simulink model "BESS_PV_WIND_STAGE2_R2_1_READABLE"  (R2026a)
settings: Solver=ode23t  StopTime=1.2  MaxStep=1e-5
InitFcn:
  | run(fullfile(fileparts(get_param(bdroot,'FileName')),'..','scripts','init_bess_pv_wind_stage2_r1.m'));
undefined symbols (not defined in the file): Control, G, S1, S2, S21, S2_API, W1
libraries: ee_lib x27, nesl_utility x23, fl_lib x10, simulink x4, sl_discontinuities x1
(part 2 of 2)

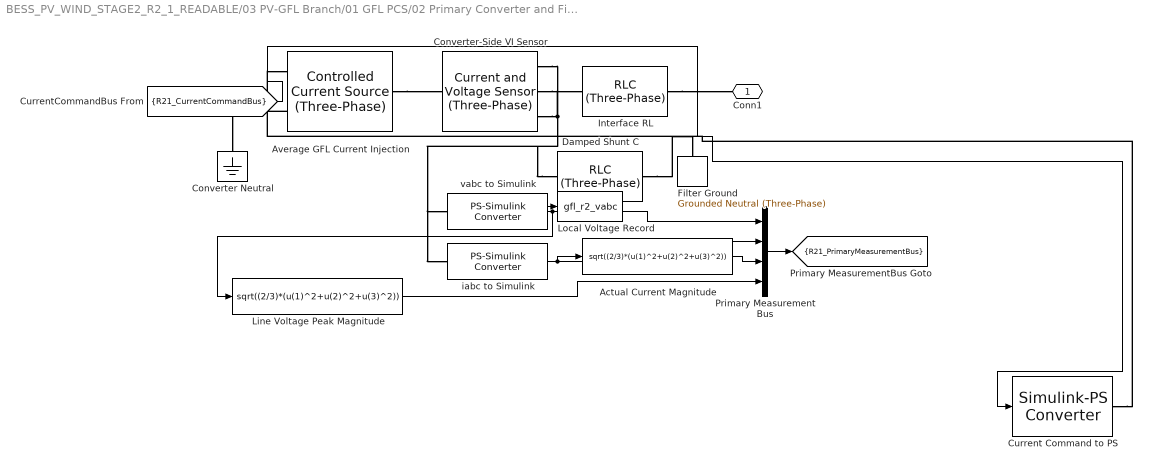
== system BESS_PV_WIND_STAGE2_R2_1_READABLE/03 PV-GFL Branch/01 GFL PCS/02 Primary Converter and Filter ==
  Actual Current Magnitude : Fcn  Expr=sqrt((2/3)*(u(1)^2+u(2)^2+u(3)^2))
  Average GFL Current Injection : ee_lib/Sources/Controlled Current Source (Three-Phase)  port_option=ee.enum.threePhasePort.composite  input_option=ee.enum.inputType.instantaneous  FRated=S1.base.f_Hz Hz  G_parasitic=1e-6 1/Ohm
  Converter Neutral : fl_lib/Electrical/Electrical Elements/Electrical Reference
  Converter-Side VI Sensor : ee_lib/Sensors & Transducers/Current and Voltage Sensor (Three-Phase)  port_option=ee.enum.threePhasePort.composite  vMeasurementType=ee.enum.vmeasurement.ll  outputUnit=ee.enum.unit.si  SRated=100e6 A*V  VRated=24e3 V  I_specify=off  I_priority=None  I=[0, 0, 0] A  I_nominal_specify=off  I_nominal_value=1  I_nominal_unit=A  V_specify=off  V_priority=None  V=[0, 0, 0] V  V_nominal_specify=off  V_nominal_value=1  V_nominal_unit=V
  Current Command to PS : nesl_utility/Simulink-PS Converter  PhysicalDomain=network_engine_domain  SubClassName=ps_input  LeftPortType=input  RightPortType=output  PseudoPeriodic=off  Frequencies=[]  NoiseDistribution=none  NoiseParameters=[]  Unit=A  AffineConversion=off  FilteringAndDerivatives=zero  SimscapeFilterOrder=1  InputFilterTimeConstant=0.001  UdotUserProvided=0
  Damped Shunt C : ee_lib/Passive/RLC Assemblies/RLC (Three-Phase)  port_option=ee.enum.threePhasePort.composite  component_structure=ee.enum.rlc.structure.SeriesRC  R=S1.filter.Rd_ohm Ohm  L=1e-3 H  C=S1.filter.C_F F  R_parasitic=0 Ohm  G_parasitic=0 1/Ohm  IL_specify=off  IL_priority=High  IL=[0, 0, 0] A  IL_nominal_specify=off  IL_nominal_value=1  IL_nominal_unit=A  VC_specify=off  VC_priority=High  VC=[0, 0, 0] V  VC_nominal_specify=off  VC_nominal_value=1  VC_nominal_unit=V
  Filter Ground : ee_lib/Connectors & References/Grounded Neutral (Three-Phase)  port_option=ee.enum.threePhasePort.composite
  Interface RL : ee_lib/Passive/RLC Assemblies/RLC (Three-Phase)  port_option=ee.enum.threePhasePort.composite  component_structure=ee.enum.rlc.structure.R  R=S1.filter.R1_ohm+S1.filter.R2_ohm Ohm  L=1e-3 H  C=1e-6 F  R_parasitic=0 Ohm  G_parasitic=0 1/Ohm  IL_specify=off  IL_priority=High  IL=[0, 0, 0] A  IL_nominal_specify=off  IL_nominal_value=1  IL_nominal_unit=A  VC_specify=off  VC_priority=High  VC=[0, 0, 0] V  VC_nominal_specify=off  VC_nominal_value=1  VC_nominal_unit=V
  Line Voltage Peak Magnitude : Fcn  Expr=sqrt((2/3)*(u(1)^2+u(2)^2+u(3)^2))
  Local Voltage Record : ToWorkspace  VariableName=gfl_r2_vabc  SampleTime=-1
  Primary MeasurementBus : Mux
  iabc to Simulink : nesl_utility/PS-Simulink Converter  PhysicalDomain=network_engine_domain  SubClassName=ps_output  LeftPortType=input  RightPortType=output  PseudoPeriodic=off  Frequencies=[]  VectorFormat=inherit  Unit=A  AffineConversion=off
  vabc to Simulink : nesl_utility/PS-Simulink Converter  PhysicalDomain=network_engine_domain  SubClassName=ps_output  LeftPortType=input  RightPortType=output  PseudoPeriodic=off  Frequencies=[]  VectorFormat=inherit  Unit=V  AffineConversion=off
  Conn1 : PMIOPort  Side=Right
  tag scope: R21_PrimaryMeasurementBus=scoped
  wires:
  iabc to Simulink/1 -> Primary MeasurementBus/2, Actual Current Magnitude/1
  vabc to Simulink/1 -> Primary MeasurementBus/1, Line Voltage Peak Magnitude/1, Local Voltage Record/1
  [R21_CurrentCommandBus] -> Current Command to PS/1
  Primary MeasurementBus/1 -> [R21_PrimaryMeasurementBus]
  Actual Current Magnitude/1 -> Primary MeasurementBus/3
  Line Voltage Peak Magnitude/1 -> Primary MeasurementBus/4
  connections:
  Damped Shunt C/LConn1 -- Converter-Side VI Sensor/RConn3 -- Interface RL/LConn1
  Current Command to PS/RConn1 -- Average GFL Current Injection/LConn1
  Converter-Side VI Sensor/RConn1 -- vabc to Simulink/LConn1
  Average GFL Current Injection/LConn2 -- Converter Neutral/LConn1
  Interface RL/RConn1 -- Conn1/RConn1
  Converter-Side VI Sensor/RConn2 -- iabc to Simulink/LConn1
  Damped Shunt C/RConn1 -- Filter Ground/LConn1
  Average GFL Current Injection/RConn1 -- Converter-Side VI Sensor/LConn1

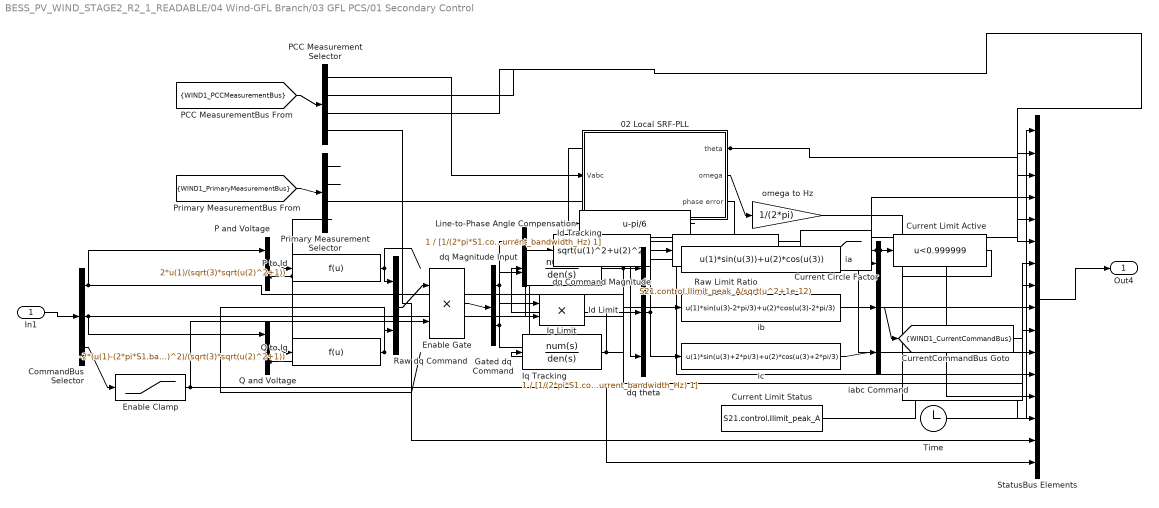
== system BESS_PV_WIND_STAGE2_R2_1_READABLE/04 Wind-GFL Branch/03 GFL PCS/01 Secondary Control ==
  In1 : Inport
  02 Local SRF-PLL : Subsystem
      settings: AttributesFormatString=|
      | local abc voltage only
      | wrapped phase-error PI
  CommandBus Selector : Demux  Outputs=3
  Current Circle Factor : Saturate  UpperLimit=1  LowerLimit=0
  Current Limit Active : Fcn  Expr=u<0.999999
  Current Limit Status : Constant  Value=S21.control.Ilimit_peak_A
  Enable Clamp : Saturate  UpperLimit=1  LowerLimit=0
  Enable Gate : Product  Inputs=**
  Gated dq Command : Demux  Outputs=2
  Id Limit : Product  Inputs=**
  Id Tracking : TransferFcn  Numerator=1  Denominator=[1/(2*pi*S1.control.current_bandwidth_Hz) 1]
  Iq Limit : Product  Inputs=**
  Iq Tracking : TransferFcn  Numerator=1  Denominator=[1/(2*pi*S1.control.current_bandwidth_Hz) 1]
  Line-to-Phase Angle Compensation : Fcn  Expr=u-pi/6
  P and Voltage : Mux  Inputs=2
  P to Id : Fcn  Expr=2*u(1)/(sqrt(3)*sqrt(u(2)^2+1))
  PCC Measurement Selector : Demux  Outputs=[3 1 1 1]
  Primary Measurement Selector : Demux  Outputs=[3 3 1 1]
  Q and Voltage : Mux  Inputs=2
  Q to Iq : Fcn  Expr=-2*(u(1)-(2*pi*S1.base.f_Hz*S1.filter.C_F/2)*u(2)^2)/(sqrt(3)*sqrt(u(2)^2+1))
  Raw Limit Ratio : Fcn  Expr=S21.control.Ilimit_peak_A/sqrt(u^2+1e-12)
  Raw dq Command : Mux  Inputs=2
  StatusBus Elements : Mux  Inputs=16
  Time : Clock
  dq Command Magnitude : Fcn  Expr=sqrt(u(1)^2+u(2)^2)
  dq Magnitude Input : Mux  Inputs=2
  dq theta : Mux  Inputs=3
  ia : Fcn  Expr=u(1)*sin(u(3))+u(2)*cos(u(3))
  iabc Command : Mux  Inputs=3
  ib : Fcn  Expr=u(1)*sin(u(3)-2*pi/3)+u(2)*cos(u(3)-2*pi/3)
  ic : Fcn  Expr=u(1)*sin(u(3)+2*pi/3)+u(2)*cos(u(3)+2*pi/3)
  omega to Hz : Gain  Gain=1/(2*pi)
  Out4 : Outport
  tag scope: WIND1_CurrentCommandBus=scoped
  wires:
  dq Command Magnitude/1 -> Raw Limit Ratio/1
  Current Limit Status/1 -> StatusBus Elements/10
  StatusBus Elements/1 -> Out4/1
  Enable Gate/1 -> Gated dq Command/1
  Q to Iq/1 -> Raw dq Command/2
  [WIND1_PrimaryMeasurementBus] -> Primary Measurement Selector/1
  Id Limit/1 -> Id Tracking/1
  PCC Measurement Selector/2 -> StatusBus Elements/2
  CommandBus Selector/2 -> StatusBus Elements/5, Q and Voltage/1
  02 Local SRF-PLL/2(omega) -> omega to Hz/1
  ib/1 -> iabc Command/2
  02 Local SRF-PLL/1(theta) -> StatusBus Elements/6, Line-to-Phase Angle Compensation/1
  Primary Measurement Selector/2 -> ?
  Primary Measurement Selector/3 -> StatusBus Elements/12
  ic/1 -> iabc Command/3
  Primary Measurement Selector/1 -> ?
  Time/1 -> StatusBus Elements/1
  Raw Limit Ratio/1 -> Current Circle Factor/1
  Current Circle Factor/1 -> Iq Limit/2, Id Limit/2, StatusBus Elements/13, Current Limit Active/1
  iabc Command/1 -> [WIND1_CurrentCommandBus]
  Gated dq Command/2 -> Iq Limit/1, dq Magnitude Input/2
  CommandBus Selector/1 -> StatusBus Elements/4, P and Voltage/1
  PCC Measurement Selector/3 -> StatusBus Elements/3
  omega to Hz/1 -> StatusBus Elements/7
  Raw dq Command/1 -> Enable Gate/1
  Gated dq Command/1 -> Id Limit/1, dq Magnitude Input/1
  Primary Measurement Selector/4 -> Q and Voltage/2, P and Voltage/2
  dq theta/1 -> ic/1, ib/1, ia/1
  Iq Tracking/1 -> StatusBus Elements/9, dq theta/2
  CommandBus Selector/3 -> Enable Clamp/1
  Enable Clamp/1 -> StatusBus Elements/16, Enable Gate/2
  In1/1 -> CommandBus Selector/1
  Id Tracking/1 -> StatusBus Elements/8, dq theta/1
  [WIND1_PCCMeasurementBus] -> PCC Measurement Selector/1
  P to Id/1 -> Raw dq Command/1
  Q and Voltage/1 -> Q to Iq/1
  PCC Measurement Selector/1 -> 02 Local SRF-PLL/1(Vabc)
  02 Local SRF-PLL/3(phase error) -> StatusBus Elements/11
  Current Limit Active/1 -> StatusBus Elements/14
  Iq Limit/1 -> Iq Tracking/1
  ia/1 -> iabc Command/1
  Line-to-Phase Angle Compensation/1 -> dq theta/3
  P and Voltage/1 -> P to Id/1
  dq Magnitude Input/1 -> dq Command Magnitude/1
  PCC Measurement Selector/4 -> StatusBus Elements/15

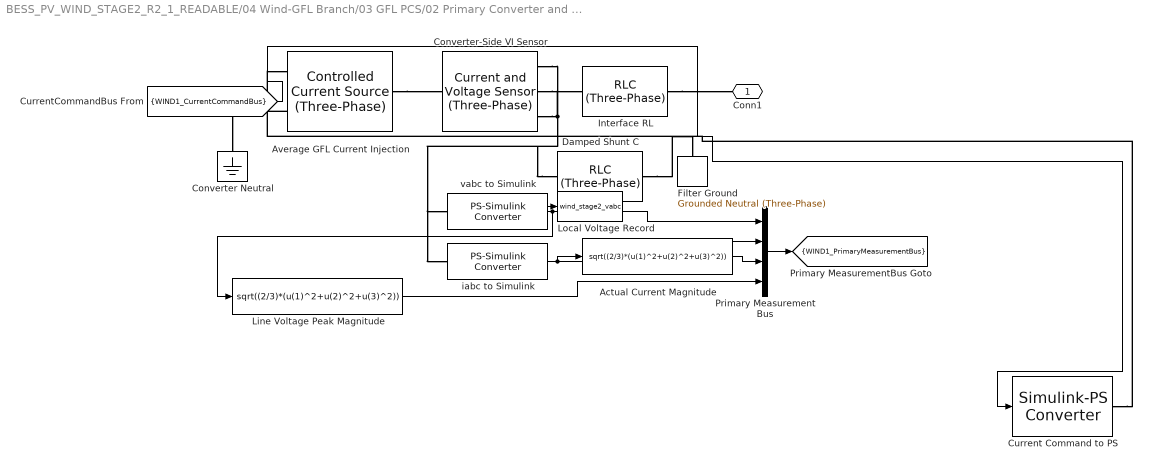
== system BESS_PV_WIND_STAGE2_R2_1_READABLE/04 Wind-GFL Branch/03 GFL PCS/02 Primary Converter and Filter ==
  Actual Current Magnitude : Fcn  Expr=sqrt((2/3)*(u(1)^2+u(2)^2+u(3)^2))
  Average GFL Current Injection : ee_lib/Sources/Controlled Current Source (Three-Phase)  port_option=ee.enum.threePhasePort.composite  input_option=ee.enum.inputType.instantaneous  FRated=S1.base.f_Hz Hz  G_parasitic=1e-6 1/Ohm
  Converter Neutral : fl_lib/Electrical/Electrical Elements/Electrical Reference
  Converter-Side VI Sensor : ee_lib/Sensors & Transducers/Current and Voltage Sensor (Three-Phase)  port_option=ee.enum.threePhasePort.composite  vMeasurementType=ee.enum.vmeasurement.ll  outputUnit=ee.enum.unit.si  SRated=100e6 A*V  VRated=24e3 V  I_specify=off  I_priority=None  I=[0, 0, 0] A  I_nominal_specify=off  I_nominal_value=1  I_nominal_unit=A  V_specify=off  V_priority=None  V=[0, 0, 0] V  V_nominal_specify=off  V_nominal_value=1  V_nominal_unit=V
  Current Command to PS : nesl_utility/Simulink-PS Converter  PhysicalDomain=network_engine_domain  SubClassName=ps_input  LeftPortType=input  RightPortType=output  PseudoPeriodic=off  Frequencies=[]  NoiseDistribution=none  NoiseParameters=[]  Unit=A  AffineConversion=off  FilteringAndDerivatives=zero  SimscapeFilterOrder=1  InputFilterTimeConstant=0.001  UdotUserProvided=0
  Damped Shunt C : ee_lib/Passive/RLC Assemblies/RLC (Three-Phase)  port_option=ee.enum.threePhasePort.composite  component_structure=ee.enum.rlc.structure.SeriesRC  R=S1.filter.Rd_ohm Ohm  L=1e-3 H  C=S1.filter.C_F F  R_parasitic=0 Ohm  G_parasitic=0 1/Ohm  IL_specify=off  IL_priority=High  IL=[0, 0, 0] A  IL_nominal_specify=off  IL_nominal_value=1  IL_nominal_unit=A  VC_specify=off  VC_priority=High  VC=[0, 0, 0] V  VC_nominal_specify=off  VC_nominal_value=1  VC_nominal_unit=V
  Filter Ground : ee_lib/Connectors & References/Grounded Neutral (Three-Phase)  port_option=ee.enum.threePhasePort.composite
  Interface RL : ee_lib/Passive/RLC Assemblies/RLC (Three-Phase)  port_option=ee.enum.threePhasePort.composite  component_structure=ee.enum.rlc.structure.R  R=S1.filter.R1_ohm+S1.filter.R2_ohm Ohm  L=1e-3 H  C=1e-6 F  R_parasitic=0 Ohm  G_parasitic=0 1/Ohm  IL_specify=off  IL_priority=High  IL=[0, 0, 0] A  IL_nominal_specify=off  IL_nominal_value=1  IL_nominal_unit=A  VC_specify=off  VC_priority=High  VC=[0, 0, 0] V  VC_nominal_specify=off  VC_nominal_value=1  VC_nominal_unit=V
  Line Voltage Peak Magnitude : Fcn  Expr=sqrt((2/3)*(u(1)^2+u(2)^2+u(3)^2))
  Local Voltage Record : ToWorkspace  VariableName=wind_stage2_vabc  SampleTime=-1
  Primary MeasurementBus : Mux
  iabc to Simulink : nesl_utility/PS-Simulink Converter  PhysicalDomain=network_engine_domain  SubClassName=ps_output  LeftPortType=input  RightPortType=output  PseudoPeriodic=off  Frequencies=[]  VectorFormat=inherit  Unit=A  AffineConversion=off
  vabc to Simulink : nesl_utility/PS-Simulink Converter  PhysicalDomain=network_engine_domain  SubClassName=ps_output  LeftPortType=input  RightPortType=output  PseudoPeriodic=off  Frequencies=[]  VectorFormat=inherit  Unit=V  AffineConversion=off
  Conn1 : PMIOPort  Side=Right
  tag scope: WIND1_PrimaryMeasurementBus=scoped
  wires:
  iabc to Simulink/1 -> Primary MeasurementBus/2, Actual Current Magnitude/1
  vabc to Simulink/1 -> Primary MeasurementBus/1, Line Voltage Peak Magnitude/1, Local Voltage Record/1
  [WIND1_CurrentCommandBus] -> Current Command to PS/1
  Primary MeasurementBus/1 -> [WIND1_PrimaryMeasurementBus]
  Actual Current Magnitude/1 -> Primary MeasurementBus/3
  Line Voltage Peak Magnitude/1 -> Primary MeasurementBus/4
  connections:
  Damped Shunt C/LConn1 -- Converter-Side VI Sensor/RConn3 -- Interface RL/LConn1
  Current Command to PS/RConn1 -- Average GFL Current Injection/LConn1
  Converter-Side VI Sensor/RConn1 -- vabc to Simulink/LConn1
  Average GFL Current Injection/LConn2 -- Converter Neutral/LConn1
  Interface RL/RConn1 -- Conn1/RConn1
  Converter-Side VI Sensor/RConn2 -- iabc to Simulink/LConn1
  Damped Shunt C/RConn1 -- Filter Ground/LConn1
  Average GFL Current Injection/RConn1 -- Converter-Side VI Sensor/LConn1

== system BESS_PV_WIND_STAGE2_R2_1_READABLE/06 Coordination and Monitoring/06 Supervision and Results/01 PV Command Profile ==
  CommandBus : Mux  Inputs=3
  Enable : Sum  Inputs=+++
  Enable Base : Constant
  Enable Off : Step  Time=10  FinalValue=0  SampleTime=0
  Enable On : Step  Time=11  FinalValue=0  SampleTime=0
  P Base Limit : Saturate  UpperLimit=S1.pv.P_initial_W  LowerLimit=0
  P Command : Sum
  P Increment : Step  Time=S1.pv.P_step_time_s  FinalValue=S1.pv.P_final_W-S1.pv.P_initial_W  SampleTime=0
  P Soft Start : simulink/Sources/Ramp  slope=S1.pv.P_ramp_W_per_s  start=0  InitialOutput=0
  Q Base Command : Constant  Value=S1.pv.Q_ref_var
  Q Command : Sum
  Q Increment : Step  Time=S1.pv.P_step_time_s  FinalValue=0  SampleTime=0
  CommandBus Out : Outport
  wires:
  Enable/1 -> CommandBus/3
  Enable On/1 -> Enable/3
  Enable Off/1 -> Enable/2
  Enable Base/1 -> Enable/1
  CommandBus/1 -> CommandBus Out/1
  Q Command/1 -> CommandBus/2
  P Command/1 -> CommandBus/1
  Q Increment/1 -> Q Command/2
  Q Base Command/1 -> Q Command/1
  P Increment/1 -> P Command/2
  P Base Limit/1 -> P Command/1
  P Soft Start/1 -> P Base Limit/1

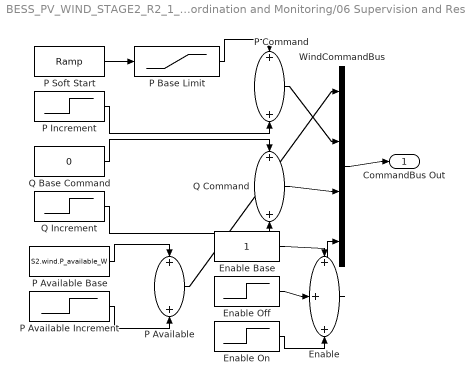
== system BESS_PV_WIND_STAGE2_R2_1_READABLE/06 Coordination and Monitoring/06 Supervision and Results/02 Wind Command Profile ==
  Enable : Sum  Inputs=+++
  Enable Base : Constant
  Enable Off : Step  Time=10  FinalValue=0  SampleTime=0
  Enable On : Step  Time=11  FinalValue=0  SampleTime=0
  P Available : Sum
  P Available Base : Constant  Value=S2.wind.P_available_W
  P Available Increment : Step  Time=S2.event_time_s  FinalValue=0  SampleTime=0
  P Base Limit : Saturate  UpperLimit=S2.wind.P_base_W  LowerLimit=0
  P Command : Sum
  P Increment : Step  Time=S2.event_time_s  FinalValue=S2.wind.P_step_W  SampleTime=0
  P Soft Start : simulink/Sources/Ramp  slope=S1.pv.P_ramp_W_per_s  start=0  InitialOutput=0
  Q Base Command : Constant  Value=0
  Q Command : Sum
  Q Increment : Step  Time=W1.command.Q_step_time_s  FinalValue=0  SampleTime=0
  WindCommandBus : Mux
  CommandBus Out : Outport
  wires:
  Enable/1 -> WindCommandBus/4
  Q Command/1 -> WindCommandBus/3
  P Command/1 -> WindCommandBus/2
  P Available/1 -> WindCommandBus/1
  P Available Increment/1 -> P Available/2
  P Available Base/1 -> P Available/1
  Enable On/1 -> Enable/3
  Enable Off/1 -> Enable/2
  Enable Base/1 -> Enable/1
  WindCommandBus/1 -> CommandBus Out/1
  Q Increment/1 -> Q Command/2
  Q Base Command/1 -> Q Command/1
  P Increment/1 -> P Command/2
  P Base Limit/1 -> P Command/1
  P Soft Start/1 -> P Base Limit/1

== system BESS_PV_WIND_STAGE2_R2_1_READABLE/03 PV-GFL Branch/01 GFL PCS/01 Secondary Control/02 Local SRF-PLL ==
  Vabc : Inport
  Angle Integrator : Integrator  InitialCondition=Control.PLL.Theta0
  Delta Omega : Sum
  Error Integral : Integrator
  Measured Phase : Fcn  Expr=atan2((2/3)*(u(1)-0.5*u(2)-0.5*u(3)),(sqrt(3)/3)*(u(3)-u(2)))
  Nominal Omega : Constant  Value=Control.PLL.OmegaNominal
  Omega Command : Sum
  Omega Limits : Saturate  UpperLimit=Control.PLL.OmegaMax  LowerLimit=Control.PLL.OmegaMin
  PLL Ki : Gain  Gain=Control.PLL.Ki
  PLL Kp : Gain  Gain=Control.PLL.Kp
  Phase Pair : Mux  Inputs=2
  Wrapped Phase Error : Fcn  Expr=atan2(sin(u(1)-u(2)),cos(u(1)-u(2)))
  theta : Outport
  omega : Outport  Port=2
  phase error : Outport  Port=3
  wires:
  Omega Limits/1 -> omega/1, Angle Integrator/1
  Omega Command/1 -> Omega Limits/1
  Nominal Omega/1 -> Omega Command/2
  Delta Omega/1 -> Omega Command/1
  Error Integral/1 -> Delta Omega/2
  PLL Kp/1 -> Delta Omega/1
  PLL Ki/1 -> Error Integral/1
  Wrapped Phase Error/1 -> phase error/1, PLL Ki/1, PLL Kp/1
  Phase Pair/1 -> Wrapped Phase Error/1
  Angle Integrator/1 -> theta/1, Phase Pair/2
  Measured Phase/1 -> Phase Pair/1
  Vabc/1 -> Measured Phase/1

== system BESS_PV_WIND_STAGE2_R2_1_READABLE/04 Wind-GFL Branch/03 GFL PCS/01 Secondary Control/02 Local SRF-PLL ==
  Vabc : Inport
  Angle Integrator : Integrator  InitialCondition=Control.PLL.Theta0
  Delta Omega : Sum
  Error Integral : Integrator
  Measured Phase : Fcn  Expr=atan2((2/3)*(u(1)-0.5*u(2)-0.5*u(3)),(sqrt(3)/3)*(u(3)-u(2)))
  Nominal Omega : Constant  Value=Control.PLL.OmegaNominal
  Omega Command : Sum
  Omega Limits : Saturate  UpperLimit=Control.PLL.OmegaMax  LowerLimit=Control.PLL.OmegaMin  ZeroCross=off
  PLL Ki : Gain  Gain=Control.PLL.Ki
  PLL Kp : Gain  Gain=Control.PLL.Kp
  Phase Pair : Mux  Inputs=2
  Wrapped Phase Error : Fcn  Expr=atan2(sin(u(1)-u(2)),cos(u(1)-u(2)))
  theta : Outport
  omega : Outport  Port=2
  phase error : Outport  Port=3
  wires:
  Omega Limits/1 -> omega/1, Angle Integrator/1
  Omega Command/1 -> Omega Limits/1
  Nominal Omega/1 -> Omega Command/2
  Delta Omega/1 -> Omega Command/1
  Error Integral/1 -> Delta Omega/2
  PLL Kp/1 -> Delta Omega/1
  PLL Ki/1 -> Error Integral/1
  Wrapped Phase Error/1 -> phase error/1, PLL Ki/1, PLL Kp/1
  Phase Pair/1 -> Wrapped Phase Error/1
  Angle Integrator/1 -> theta/1, Phase Pair/2
  Measured Phase/1 -> Phase Pair/1
  Vabc/1 -> Measured Phase/1

== matlab function BESS_PV_WIND_STAGE2_R2_1_READABLE/06 Coordination and Monitoring/07 Resource API Layer/MATLAB Function Coordinator ==
  data: bess input size=[1 15]; pvCmdOut output size=[1 3]; pv input size=[1 16]; wind input size=[1 21]; pvLegacy input size=[1 3]; windLegacy input size=[1 4]; coordEnable input size=1; modes input size=[1 3]; bessDesired input size=[1 3]; config input size=[1 11]; windCmdOut output size=[1 4]; apiLog output size=[1 48]
function [pvCmdOut,windCmdOut,apiLog] = f(bess,pv,wind,pvLegacy,windLegacy,coordEnable,modes,bessDesired,config)
%#codegen
pvCmdOut=zeros(1,3); windCmdOut=zeros(1,4); apiLog=zeros(1,48);
status=zeros(3,12);
status(1,:)=[bess(2) bess(3) pv(15) bess(4) 5e6 5e6-abs(bess(2)) bess(14) 1 bess(6) bess(7) 0 5e6];
status(2,:)=[pv(2) pv(3) pv(15) pv(7) 5e6 5e6-pv(2) pv(13) 1 -1 -1 -1 5e6];
status(3,:)=[wind(2) wind(3) wind(15) wind(7) wind(17) max(0,wind(17)-wind(2)) wind(13) 1 wind(20)/1500 wind(20) wind(21) wind(18)];
cmd=[bessDesired(1) bessDesired(2) bessDesired(3) modes(1); pvLegacy(1) pvLegacy(2) pvLegacy(3) modes(2); windLegacy(2) windLegacy(3) windLegacy(4) modes(3)];
commandOut=stage2_coordinator_algorithm(status,cmd,coordEnable,config);
pvCmdOut=commandOut(2,1:3); windCmdOut=[windLegacy(1) commandOut(3,1:3)];
apiLog=[reshape(commandOut.',1,12) reshape(status.',1,36)];
end
